simulink model "SLX_Banthia"  (R2026b)
settings: Solver=VariableStepAuto
PreLoadFcn:
  | ABS_parameter
InitFcn:
  | ABS_parameter
values from neighbouring files (symbols this model uses):
  g = 9.81    [ABS_parameter.m]
  J = 1.00    (= 1)    [ABS_parameter.m]
  m = 200    [ABS_parameter.m]
  R = 0.30    (= 0.3)    [ABS_parameter.m]
  v0 = 25    [ABS_parameter.m]
settings Model: Creator=abant  LastModifiedBy=abant
settings RTWCC: GPUComputeCapability=5.0

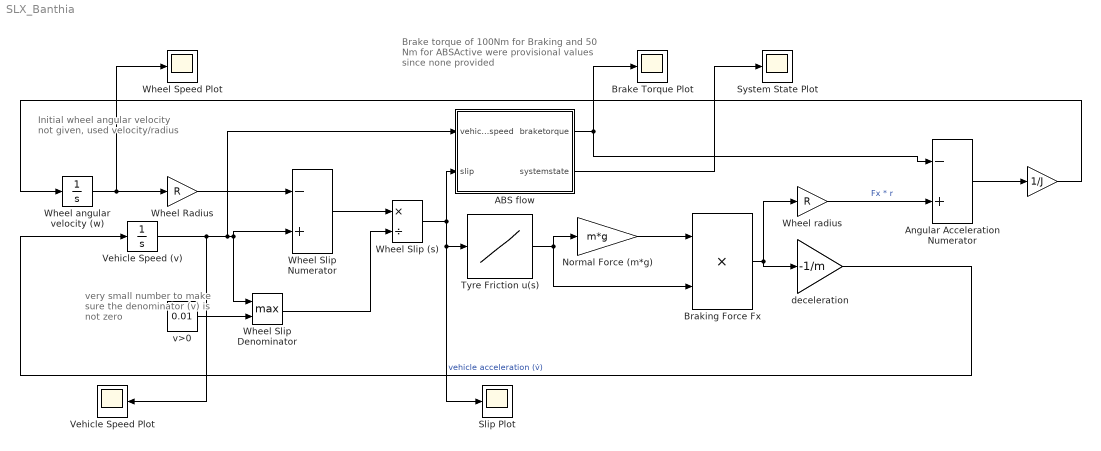
== system SLX_Banthia ==
  note: Brake torque of 100Nm for Braking and 50 Nm for ABSActive were provisional values since none provided
  note: very small number to make sure the denominator (v) is not zero
  note: Initial wheel angular velocity not given, used velocity/radius
  " " : Gain  Gain=1/J
  ABS flow : Stateflow chart  TreatAsAtomicUnit=on
  Angular Acceleration Numerator : Sum  Inputs=-+
  Brake Torque Plot : Scope
      settings: ActiveDisplayYMinimum=-12.499999999999996  ActiveDisplayYMaximum=112.5  DataLoggingVariableName=ScopeData3
  Braking Force Fx : Product
  Normal Force (m*g) : Gain  Gain=m*g
  Slip Plot : Scope
      settings: ActiveDisplayYMinimum=-0.0052876043409396415  ActiveDisplayYMaximum=0.04758843906845537  DataLoggingVariableName=ScopeData2
  System State Plot : Scope
      settings: ActiveDisplayYMinimum=-0.12499999999999997  ActiveDisplayYMaximum=1.125  DataLoggingVariableName=ScopeData4
  "Tyre Friction u(s) " : Lookup_n-D  NumberOfTableDimensions=1  BreakpointsForDimension1=[0 0.05 0.10 0.15 0.20 0.30 0.50 1.0]  Table=[0 0.60 0.90 1.00 0.95 0.75 0.40 0.10]  InternalRulePriority=Speed  RndMeth=Simplest
  Vehicle Speed (v) : Integrator  InitialCondition=v0  LimitOutput=on  LowerSaturationLimit=0
  Vehicle Speed Plot : Scope
      settings: ActiveDisplayYMinimum=8.0640425021405555  ActiveDisplayYMaximum=26.881773055317716
  Wheel Radius : Gain  Gain=R
  Wheel Slip (s) : Product  Inputs=*/
  Wheel Slip Denominator : MinMax  Function=max  Inputs=2
  "Wheel Slip Numerator " : Sum  Inputs=-+
  Wheel Speed Plot : Scope
      settings: ActiveDisplayYMinimum=25.674915523426876  ActiveDisplayYMaximum=89.739824201100731
  Wheel angular velocity (w) : Integrator  InitialCondition=v0/R  LimitOutput=on  LowerSaturationLimit=0
  Wheel radius : Gain  Gain=R
  deceleration : Gain  Gain=-1/m
  v>0 : Constant  Value=0.01
  wires:
  Wheel angular velocity (w)/1 -> Wheel Speed Plot/1, Wheel Radius/1
  Wheel Radius/1 -> "Wheel Slip Numerator "/1
  Vehicle Speed (v)/1 -> Vehicle Speed Plot/1, ABS flow/1(vehiclespeed), Wheel Slip Denominator/1, "Wheel Slip Numerator "/2
  "Tyre Friction u(s) "/1 -> Normal Force (m*g)/1, Braking Force Fx/2
  Normal Force (m*g)/1 -> Braking Force Fx/1
  v>0/1 -> Wheel Slip Denominator/2
  Wheel Slip Denominator/1 -> Wheel Slip (s)/2
  "Wheel Slip Numerator "/1 -> Wheel Slip (s)/1
  Wheel Slip (s)/1 -> Slip Plot/1, "Tyre Friction u(s) "/1, ABS flow/2(slip)
  Braking Force Fx/1 -> Wheel radius/1, deceleration/1
  deceleration/1 -> Vehicle Speed (v)/1  "vehicle acceleration (v̇)"
  Wheel radius/1 -> Angular Acceleration Numerator/2  "Fx * r"
  Angular Acceleration Numerator/1 -> " "/1
  " "/1 -> Wheel angular velocity (w)/1
  ABS flow/1(braketorque) -> Brake Torque Plot/1, Angular Acceleration Numerator/1
  ABS flow/2(systemstate) -> System State Plot/1

== stateflow chart SLX_Banthia/ABS flow ==
  state Inactive
    during: braketorque = 0;
    systemstate = 0;
  state Braking
    during: braketorque = 100;
    systemstate =1;
  state ABSActive
    during:braketorque=50;
    systemstate=2;
  (default) -> Inactive
  Braking -> ABSActive [order 1] : [slip>0.15]
  Inactive -> Braking : [vehiclespeed>10]
  ABSActive -> Braking : [slip<0.10]
  Braking -> Inactive [order 2] : [vehiclespeed<=10]
  data: vehiclespeed input double; slip input double; braketorque output double; systemstate output double
